simulink model "Battery_Energy_Storage_System"  (R2024b)
settings: Solver=FixedStepAuto  StartTime=0.0  StopTime=24  FixedStep=5e-7  RelTol=1e-3
undefined symbols (not defined in the file): Ion, Lithium
libraries: spsSeriesRLCBranchLib x6, spsCurrentMeasurementLib x3, spsIGBTDiodeLib x2, spsPWMGeneratorDCDCLib x2, spsVoltageMeasurementLib x2, spsBatteryLib x1, spsDiodeLib x1, spsMosfetLib x1, slpidlib x1, spsPVArrayLib x1, sps_lib x1
settings Model: Creator=Admin  LastModifiedBy=Admin
settings DebuggingCC: AlgebraicLoopMsg=none

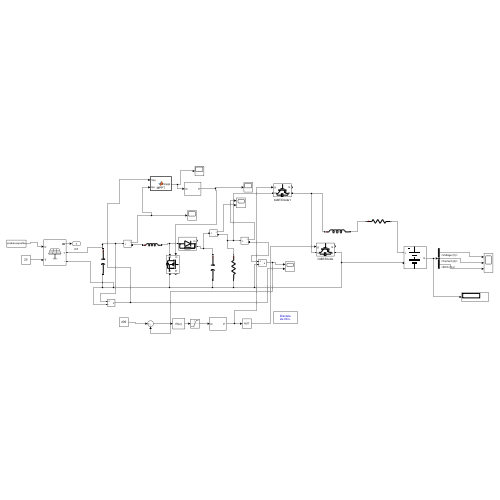
[thumbnail: Simulink's stored preview of the top-level diagram]
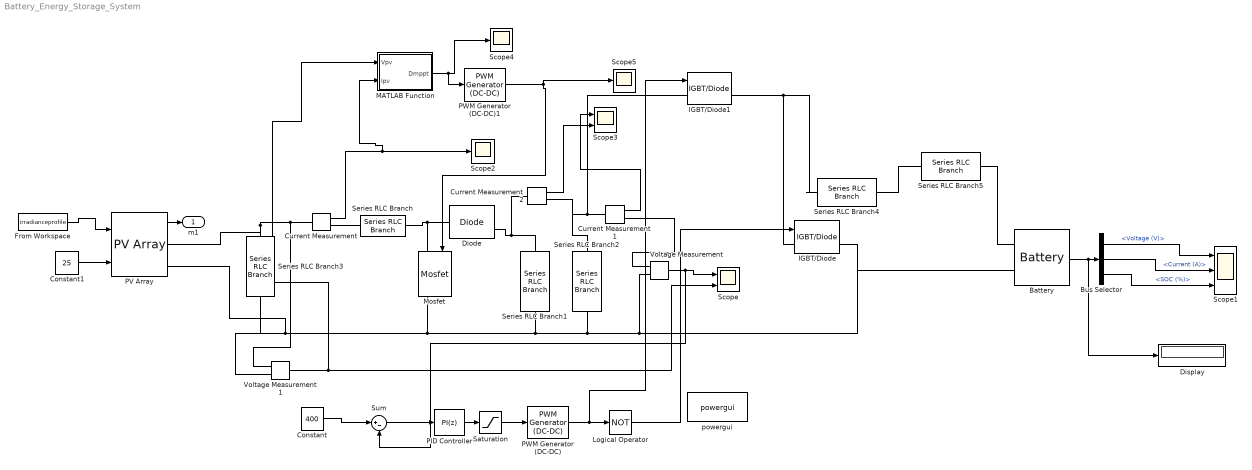
== system Battery_Energy_Storage_System ==
  Battery : spsBatteryLib/Battery  BatType=Lithium-Ion  NomV=150  NomQ=1  SOC=50  Batt_Tr=0.1  PresetModel=on  MaxQ=1  MinV=112.5  FullV=174.5981  Dis_rate=0.43478  R=1.5  Normal_OP=0.90435  expZone="[162.0579    0.04913043]"
  Bus Selector : BusSelector  OutputSignals=Voltage (V),Current (A),SOC (%)
  Constant : Constant  Value=400
  Constant1 : Constant  Value=25
  Current Measurement : spsCurrentMeasurementLib/Current Measurement  PhasorSimulation=off  OutputType=Complex  PSBequivalent=0
  Current Measurement1 : spsCurrentMeasurementLib/Current Measurement  PhasorSimulation=off  OutputType=Complex  PSBequivalent=0
  Current Measurement2 : spsCurrentMeasurementLib/Current Measurement  PhasorSimulation=off  OutputType=Complex  PSBequivalent=0
  Diode : spsDiodeLib/Diode  Ron=0.001  Lon=0  Vf=0.8  IC=0  UseSnubber=0  Rs=500  Cs=250e-9  Measurements=on
  Display : Display
  From Workspace : FromWorkspace  VariableName=irradianceprofile
  IGBT/Diode : spsIGBTDiodeLib/IGBT//Diode  Ron=1e-3  Rs=1e5  Cs=inf  Measurements=on
  IGBT/Diode1 : spsIGBTDiodeLib/IGBT//Diode  Ron=1e-3  Rs=1e5  Cs=inf  Measurements=on
  Logical Operator : Logic  Operator=NOT  AllPortsSameDT=off  OutDataTypeStr=boolean
  MATLAB Function : MATLAB Function  TreatAsAtomicUnit=on
  Mosfet : spsMosfetLib/Mosfet  Ron=0.1  Lon=0  Rd=0.01  Vfd=0  IC=0  Rs=1e5  Cs=inf  Measurements=on
  PID Controller : slpidlib/PID Controller  Controller=PI  Form=Parallel  TimeDomain=Discrete-time  UseExternalTs=off  SampleTime=5e-7  IntegratorMethod=Forward Euler  FilterMethod=Forward Euler  ControllerParametersSource=internal  P=0.01  I=1  UseKiTs=off  D=0  UseExternalDerivativeSource=off  N=100  UseFilter=on  TunerSelectOption=Transfer Function Based (PID Tuner App)  InitialConditionSource=internal  InitialConditionForIntegrator=0  InitialConditionForFilter=0  DifferentiatorICPrevScaledInput=0  ExternalReset=none  TrackingMode=off  Kt=1  LimitOutput=off  SatLimitsSource=internal  UpperSaturationLimit=inf  LowerSaturationLimit=-inf  LinearizeAsGain=on  AntiWindupMode=none  Kb=1  LimitIntegrator=off  UpperIntegratorSaturationLimit=inf  LowerIntegratorSaturationLimit=-inf  POutMin=[]  POutMax=[]  IOutMin=[]  IOutMax=[]  DOutMin=[]  DOutMax=[]  NOutMin=[]  NOutMax=[]  SumOutMin=[]  SumOutMax=[]  SaturationOutMin=[]  SaturationOutMax=[]  PParamMin=[]  PParamMax=[]  IParamMin=[]  IParamMax=[]  DParamMin=[]  DParamMax=[]  NParamMin=[]  NParamMax=[]  KbParamMin=[]  KbParamMax=[]  KtParamMin=[]  KtParamMax=[]  KbOutMin=[]  KbOutMax=[]  KtOutMin=[]  KtOutMax=[]  IntegratorOutMin=[]  IntegratorOutMax=[]  FilterOutMin=[]  FilterOutMax=[]  SumI1OutMin=[]  SumI1OutMax=[]  SumI2OutMin=[]  SumI2OutMax=[]  SumI3OutMin=[]  SumI3OutMax=[]  SumI4OutMin=[]  SumI4OutMax=[]  SumDOutMin=[]  SumDOutMax=[]  DifferentiatorOutMin=[]  DifferentiatorOutMax=[]  FilterDiffOutCoefMin=[]  FilterDiffOutCoefMax=[]  ReciprocalOutMin=[]  ReciprocalOutMax=[]  SumDenOutMin=[]  SumDenOutMax=[]  SumNumOutMin=[]  SumNumOutMax=[]  DivideOutMin=[]  DivideOutMax=[]  UdiffTsProdOutMin=[]  UdiffTsProdOutMax=[]  NTsProdOutMin=[]  NTsProdOutMax=[]  UintegralTsProdOutMin=[]  UintegralTsProdOutMax=[]  UngainTsProdOutMin=[]  UngainTsProdOutMax=[]  ClampingZeroOutDataTypeStr=Inherit: Inherit via back propagation  ClampingZeroOutMin=[]  ClampingZeroOutMax=[]  FilterDenConstantOutDataTypeStr=Inherit: Inherit via back propagation  FilterDenConstantOutMin=[]  FilterDenConstantOutMax=[]  PCopyOutDataTypeStr=Inherit: Inherit via back propagation  PCopyOutMin=[]  PCopyOutMax=[]  NCopyOutDataTypeStr=Inherit: Inherit via back propagation  NCopyOutMin=[]  NCopyOutMax=[]  IntegratorContinuousStateAttributes=''  IntegratorStateMustResolveToSignalObject=off  IntegratorRTWStateStorageClass=Auto  FilterContinuousStateAttributes=''  FilterStateMustResolveToSignalObject=off  FilterRTWStateStorageClass=Auto  ParallelPVariant=InternalParameters  IdealPVariant=Disabled  IVariant=InternalParameters  DVariant=Disabled  IntegratorVariant=Discrete  SatVariant=Disabled  AWVariant=Passthrough  PCopyVariant=Disabled  TRVariant=Disabled  FdbkBlocksVariant=Forward  IdealPFdbkVariant=Disabled  SatFdbkVariant=Disabled  DerivativeFilterVariant=Disabled  NVariant=Disabled  NCopyVariant=Disabled_SignalSpec  FilterICVariant=Disabled  IntegratorICVariant=InternalICs  ExternalResetVariant=Disabled  TRSumVariant=Passthrough  SumFdbkVariant=Disabled  SumVariant=Sum_PI  TsampFilterVariant=InternalTs  TsampNgainVariant=Passthrough  TsampIntegralVariant=Disabled_SignalSpec  ExternalSaturationOutDataTypeStr=Inherit: Same as second input  DerivativeSourceVariant=Disabled  PreIntVariant=InternalPreInt
  PV Array : spsPVArrayLib/PV Array  Npar=1  Nser=1  PlotType=array @ 1000 W/m2 & specified temperatures  S_vec="[ 1000  500  100 ]"  Temp_C_vec=[ 25]  ModuleName=User-defined  PlotWhenSelected=off  Pm=10800  Ncell=60  Voc=300  Isc=41.2  Vm=270  Im=40  beta_Voc_pc=-0.36099  alpha_Isc_pc=0.05  beta_Voc=-1.083  alpha_Isc=0.0206  IL=47.2602  I0=1.2667e-15  nI=5.1759  Rsh=14.1091  Rs=0.00084379  RobustModel=off  RobustCellTemperature=313.3991  BAL=off  Tc=1e-6  Tfilter=5e-5
  PWM Generator (DC-DC) : spsPWMGeneratorDCDCLib/PWM Generator (DC-DC)  Fsw=20000  Ts=0
  PWM Generator (DC-DC)1 : spsPWMGeneratorDCDCLib/PWM Generator (DC-DC)  Fsw=5000  Ts=0
  Saturation : Saturate  UpperLimit=0.9  LowerLimit=0.1
  Scope : Scope  NumInputPorts=2
  Scope1 : Scope  NumInputPorts=3
  Scope2 : Scope
  Scope3 : Scope  NumInputPorts=2
  Scope4 : Scope
  Scope5 : Scope
  Series RLC Branch : spsSeriesRLCBranchLib/Series RLC Branch  LConnTagsString=__new0  RConnTagsString=__new0  BranchType=L  Resistance=1  Inductance=3e-3  SetiL0=off  InitialCurrent=0  Capacitance=1e-6  Setx0=off  InitialVoltage=0  Measurements=None
  Series RLC Branch1 : spsSeriesRLCBranchLib/Series RLC Branch  LConnTagsString=__new0  RConnTagsString=__new0  BranchType=C  Resistance=1  Inductance=1e-3  SetiL0=off  InitialCurrent=0  Capacitance=500e-6  Setx0=off  InitialVoltage=0  Measurements=None
  Series RLC Branch2 : spsSeriesRLCBranchLib/Series RLC Branch  LConnTagsString=__new0  RConnTagsString=__new0  BranchType=R  Resistance=300  Inductance=1e-3  SetiL0=off  InitialCurrent=0  Capacitance=1e-6  Setx0=off  InitialVoltage=0  Measurements=None
  Series RLC Branch3 : spsSeriesRLCBranchLib/Series RLC Branch  LConnTagsString=__new0  RConnTagsString=__new0  BranchType=C  Resistance=1  Inductance=1e-3  SetiL0=off  InitialCurrent=0  Capacitance=130e-6  Setx0=off  InitialVoltage=0  Measurements=None
  Series RLC Branch4 : spsSeriesRLCBranchLib/Series RLC Branch  LConnTagsString=__new0  RConnTagsString=__new0  BranchType=L  Resistance=1  Inductance=1.81e-3  SetiL0=off  InitialCurrent=0  Capacitance=1e-6  Setx0=off  InitialVoltage=0  Measurements=None
  Series RLC Branch5 : spsSeriesRLCBranchLib/Series RLC Branch  LConnTagsString=__new0  RConnTagsString=__new0  BranchType=R  Resistance=10  Inductance=1e-3  SetiL0=off  InitialCurrent=0  Capacitance=1e-6  Setx0=off  InitialVoltage=0  Measurements=None
  Sum : Sum  Inputs=|+-
  Voltage Measurement : spsVoltageMeasurementLib/Voltage Measurement  PhasorSimulation=off  OutputType=Complex  PSBequivalent=0
  Voltage Measurement1 : spsVoltageMeasurementLib/Voltage Measurement  PhasorSimulation=off  OutputType=Complex  PSBequivalent=0
  powergui : sps_lib/powergui  Priority=1  SimulationMode=Discrete  SampleTime=2e-6  frequency=60  Iterations=50  frequencyindice=0  Pbase=100e6  ErrMax=1e-4  UnitsV=kV  UnitsW=MW  buscounter=0  FunctionMessages=off  echomessages=off  EnableUseOfTLC=off  CurrentSourceSwitches=off  DisableSnubberDevices=off  DisableRonSwitches=off  DisableVfSwitches=off  DisplayEquations=off  AutomaticDiscreteSolvers=off  SolverType=Tustin/Backward Euler (TBE)  Interpol=off  ExternalGateDelay=off  methode=off  Ts=100  x0status=blocks  SPID=on  SwTol=0  HookPort=off  NonlinearTolerance=1e-4  nMaxIteration=100  ContinueOnMaxIteration=off  RestoreLinks=warning  ResistiveCurrentMeasurement=off  Frange=[0:2:500]  Ylog=off  Xlog=on  ShowGrid=off  save=off  variable=ZData  structure=0  ZoomFFT=off  StartTime=0.0  cycles=1  DisplayStyle=1  fundamental=60  FreqAxis=off  MaxFrequency=1000  frequencyindicesteady=1  RmsSteady=1  display=off
  m1 : Outport
  wires:
  From Workspace/1 -> PV Array/1
  PV Array/1 -> m1/1
  Battery/1 -> Display/1, Bus Selector/1
  Saturation/1 -> PWM Generator (DC-DC)/1
  Voltage Measurement/1 -> Sum/2, Scope/1
  Bus Selector/1 -> Scope1/1  "<Voltage (V)>"
  Constant1/1 -> PV Array/2
  Sum/1 -> PID Controller/1
  PWM Generator (DC-DC)/1 -> IGBT/Diode1/1, Logical Operator/1
  PID Controller/1 -> Saturation/1
  Bus Selector/3 -> Scope1/3  "<SOC (%)>"
  Bus Selector/2 -> Scope1/2  "<Current (A)>"
  Voltage Measurement1/1 -> MATLAB Function/1(Vpv), Scope/2
  Current Measurement/1 -> MATLAB Function/2(Ipv), Scope2/1
  Current Measurement1/1 -> Scope3/1
  Current Measurement2/1 -> Scope3/2
  Constant/1 -> Sum/1
  PWM Generator (DC-DC)1/1 -> Mosfet/1, Scope5/1
  Logical Operator/1 -> IGBT/Diode/1
  MATLAB Function/1(Dmppt) -> PWM Generator (DC-DC)1/1, Scope4/1
  connections:
  Voltage Measurement/LConn2 -- IGBT/Diode/RConn1 -- Battery/LConn2 -- Series RLC Branch1/RConn1 -- Series RLC Branch3/RConn1 -- Voltage Measurement1/LConn2 -- PV Array/RConn2 -- Mosfet/RConn1 -- Series RLC Branch2/RConn1
  Series RLC Branch4/LConn1 -- IGBT/Diode/LConn1 -- IGBT/Diode1/RConn1
  Voltage Measurement1/LConn1 -- Current Measurement/LConn1 -- PV Array/RConn1 -- Series RLC Branch3/LConn1
  Diode/LConn1 -- Mosfet/LConn1 -- Series RLC Branch/RConn1
  Series RLC Branch5/LConn1 -- Series RLC Branch4/RConn1
  Series RLC Branch5/RConn1 -- Battery/LConn1
  Current Measurement/RConn1 -- Series RLC Branch/LConn1
  Current Measurement1/LConn1 -- Series RLC Branch2/LConn1 -- Current Measurement2/RConn1 -- IGBT/Diode1/LConn1
  Current Measurement1/RConn1 -- Voltage Measurement/LConn1
  Series RLC Branch1/LConn1 -- Current Measurement2/LConn1 -- Diode/RConn1

== matlab function Battery_Energy_Storage_System/MATLAB Function ==
  data: Vpv input; Dmppt output; Ipv input
function Dmppt = MPPT(Vpv, Ipv)
%#codegen
persistent Vprev Pprev Dprev dir cnt sumV sumI
Ts    = 1e-6;                 % powergui sample time (change if different)
Tmppt = 5e-3;                 % MPPT update period
N     = round(Tmppt/Ts);
D0    = 1 - 270/400;          % 0.325
Dmin  = 0.25;  Dmax = 0.60;
DeltaD = 0.002;

if isempty(Vprev)
    Vprev = Vpv; Pprev = Vpv*Ipv; Dprev = D0;
    dir = 1; cnt = 0; sumV = 0; sumI = 0;
end

% accumulate for averaging
sumV = sumV + Vpv;
sumI = sumI + Ipv;
cnt  = cnt + 1;

Dmppt = Dprev;

if cnt >= N
    V = sumV/cnt;  I = sumI/cnt;
    sumV = 0; sumI = 0; cnt = 0;

    P  = V*I;
    dV = V - Vprev;
    dP = P - Pprev;

    if P < 1
        % night: reset
        Dmppt = D0;
        dir = 1;
    else
        if abs(dP) > 0.0005*P
            if (dP > 0 && dV > 0) || (dP < 0 && dV < 0)
                dir = -1;     % Vpv should go up, so D down
            else
                dir = 1;      % Vpv should go down, so D up
            end
        end
        Dmppt = Dprev + dir*DeltaD;

        % at a limit, turn around instead of sticking
        if Dmppt >= Dmax
            Dmppt = Dmax; dir = -1;
        elseif Dmppt <= Dmin
            Dmppt = Dmin; dir = 1;
        end
    end

    Vprev = V; Pprev = P; Dprev = Dmppt;
end
end
